simulink model "conversaoAD"  (R2024b)
settings: Solver=VariableStepAuto  StartTime=0.0  StopTime=1  RelTol=1e-3
libraries: simulink_extras x1, simulink x1

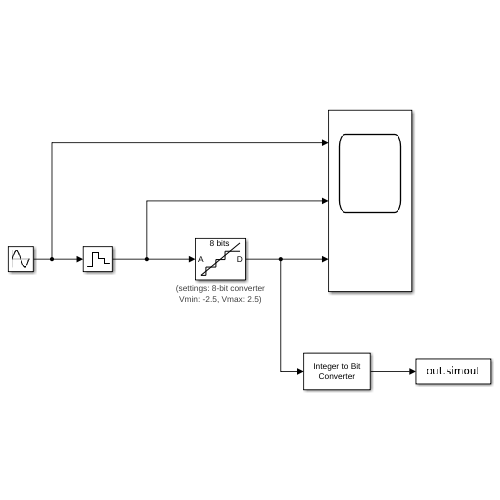
[thumbnail: Simulink's stored preview of the top-level diagram]
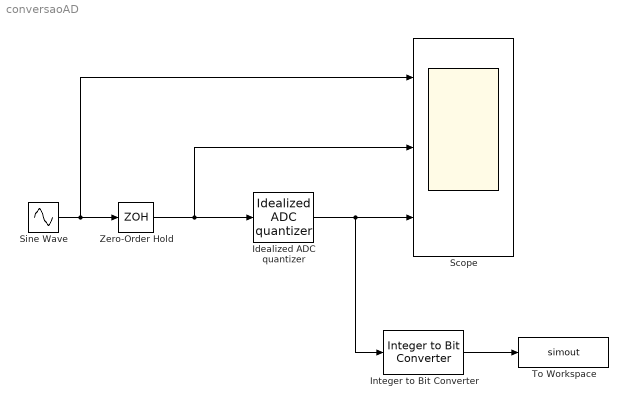
== system conversaoAD ==
  Idealized ADC quantizer : simulink_extras/Additional Discrete/Idealized ADC quantizer  NumberOfConverterBits=8  Vmin=-2.5  Vmax=2.5  OutputDataType=single  OutputNegativeValues=off
  Integer to Bit Converter : simulink/Logic and Bit Operations/Integer to Bit Converter  nbits=8  signedInputValues=Unsigned  bitOrder=MSB first  outDtype=single
  Scope : Scope  NumInputPorts=3
  Sine Wave : Sin  Amplitude=2.5  Frequency=4*pi  SampleTime=0
  To Workspace : ToWorkspace  VariableName=simout  SaveFormat=Timeseries  SampleTime=-1
  Zero-Order Hold : ZeroOrderHold  SampleTime=1/20
  wires:
  Sine Wave/1 -> Scope/1, Zero-Order Hold/1
  Zero-Order Hold/1 -> Idealized ADC quantizer/1, Scope/2
  Idealized ADC quantizer/1 -> Integer to Bit Converter/1, Scope/3
  Integer to Bit Converter/1 -> To Workspace/1
